simulink model "fullcar_7dof"  (R2026a)
settings: Solver=ode4  StopTime=t_end  FixedStep=dt
values from neighbouring files (symbols this model uses):
  Kfb = lqr(Aa, Ba, Q, R, N)    [controller_lqr.m]    (also in controller_skyhook.m = diag(c_sky) * [zeros(4, 7), veh.T, zeros(4, 4), zeros(4, 8)]; test_controllers.m = {zeros(4,22), K}; test_fullcar_model.m = K{1})
  x0 = -(A - Bu * Kfb(:, 1:14)) \ ((B(:, 5:12) - Bu * Kfb(:, 15:22)) * w(1, 2:9)')    [run_fullcar.m]    (also in test_fullcar_model.m = zeros(14,1))
undefined symbols (not defined in the file or in its folder): veh
settings Model: Creator=markn  LastModifiedBy=markn
settings DataIOCC: ExternalInput=w_in  LoadExternalInput=on
settings DebuggingCC: AlgebraicLoopMsg=error

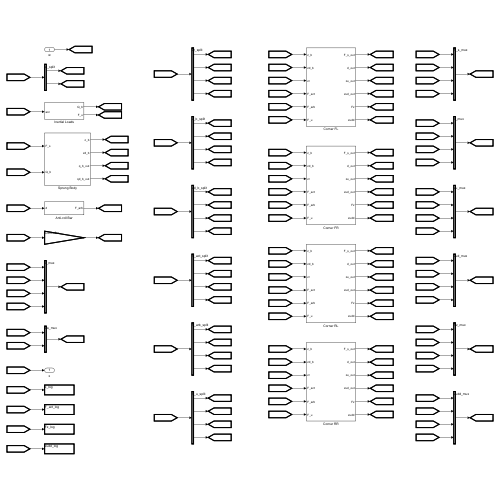
[thumbnail: Simulink's stored preview of the top-level diagram]
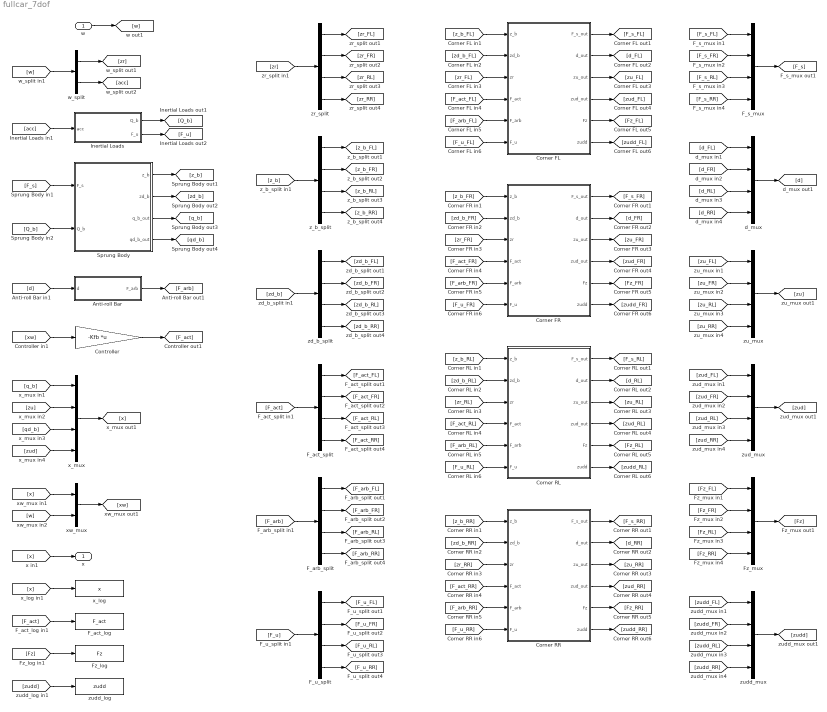
== system fullcar_7dof ==
  w : Inport  PortDimensions=8
  Anti-roll Bar : Subsystem
  Controller : Gain  Gain=-Kfb  Multiplication=Matrix(K*u)
  Corner FL : Subsystem
  Corner FR : Subsystem
  Corner RL : Subsystem
  Corner RR : Subsystem
  F_act_log : ToWorkspace  VariableName=F_act  SampleTime=-1
  F_act_split : Demux
  F_arb_split : Demux
  F_s_mux : Mux
  F_u_split : Demux
  Fz_log : ToWorkspace  VariableName=Fz  SampleTime=-1
  Fz_mux : Mux
  Inertial Loads : Subsystem
  Sprung Body : Subsystem
  d_mux : Mux
  w_split : Demux  Outputs=[4 4]
  x_log : ToWorkspace  VariableName=x  SampleTime=-1
  x_mux : Mux  Inputs=[3 4 3 4]
  xw_mux : Mux  Inputs=[14 8]
  z_b_split : Demux
  zd_b_split : Demux
  zr_split : Demux
  zu_mux : Mux
  zud_mux : Mux
  zudd_log : ToWorkspace  VariableName=zudd  SampleTime=-1
  zudd_mux : Mux
  x : Outport
  wires:
  w/1 -> [w]
  [w] -> w_split/1
  w_split/1 -> [zr]
  w_split/2 -> [acc]
  [acc] -> Inertial Loads/1(acc)
  Inertial Loads/1(Q_b) -> [Q_b]
  Inertial Loads/2(F_u) -> [F_u]
  [F_s] -> Sprung Body/1(F_s)
  [Q_b] -> Sprung Body/2(Q_b)
  Sprung Body/1(z_b) -> [z_b]
  Sprung Body/2(zd_b) -> [zd_b]
  Sprung Body/3(q_b_out) -> [q_b]
  Sprung Body/4(qd_b_out) -> [qd_b]
  [d] -> Anti-roll Bar/1(d)
  Anti-roll Bar/1(F_arb) -> [F_arb]
  [xw] -> Controller/1
  Controller/1 -> [F_act]
  [q_b] -> x_mux/1
  [zu] -> x_mux/2
  [qd_b] -> x_mux/3
  [zud] -> x_mux/4
  x_mux/1 -> [x]
  [x] -> xw_mux/1
  [w] -> xw_mux/2
  xw_mux/1 -> [xw]
  [x] -> x/1
  [x] -> x_log/1
  [F_act] -> F_act_log/1
  [Fz] -> Fz_log/1
  [zudd] -> zudd_log/1
  [zr] -> zr_split/1
  zr_split/1 -> [zr_FL]
  zr_split/2 -> [zr_FR]
  zr_split/3 -> [zr_RL]
  zr_split/4 -> [zr_RR]
  [z_b] -> z_b_split/1
  z_b_split/1 -> [z_b_FL]
  z_b_split/2 -> [z_b_FR]
  z_b_split/3 -> [z_b_RL]
  z_b_split/4 -> [z_b_RR]
  [zd_b] -> zd_b_split/1
  zd_b_split/1 -> [zd_b_FL]
  zd_b_split/2 -> [zd_b_FR]
  zd_b_split/3 -> [zd_b_RL]
  zd_b_split/4 -> [zd_b_RR]
  [F_act] -> F_act_split/1
  F_act_split/1 -> [F_act_FL]
  F_act_split/2 -> [F_act_FR]
  F_act_split/3 -> [F_act_RL]
  F_act_split/4 -> [F_act_RR]
  [F_arb] -> F_arb_split/1
  F_arb_split/1 -> [F_arb_FL]
  F_arb_split/2 -> [F_arb_FR]
  F_arb_split/3 -> [F_arb_RL]
  F_arb_split/4 -> [F_arb_RR]
  [F_u] -> F_u_split/1
  F_u_split/1 -> [F_u_FL]
  F_u_split/2 -> [F_u_FR]
  F_u_split/3 -> [F_u_RL]
  F_u_split/4 -> [F_u_RR]
  [z_b_FL] -> Corner FL/1(z_b)
  [zd_b_FL] -> Corner FL/2(zd_b)
  [zr_FL] -> Corner FL/3(zr)
  [F_act_FL] -> Corner FL/4(F_act)
  [F_arb_FL] -> Corner FL/5(F_arb)
  [F_u_FL] -> Corner FL/6(F_u)
  Corner FL/1(F_s_out) -> [F_s_FL]
  Corner FL/2(d_out) -> [d_FL]
  Corner FL/3(zu_out) -> [zu_FL]
  Corner FL/4(zud_out) -> [zud_FL]
  Corner FL/5(Fz) -> [Fz_FL]
  Corner FL/6(zudd) -> [zudd_FL]
  [z_b_FR] -> Corner FR/1(z_b)
  [zd_b_FR] -> Corner FR/2(zd_b)
  [zr_FR] -> Corner FR/3(zr)
  [F_act_FR] -> Corner FR/4(F_act)
  [F_arb_FR] -> Corner FR/5(F_arb)
  [F_u_FR] -> Corner FR/6(F_u)
  Corner FR/1(F_s_out) -> [F_s_FR]
  Corner FR/2(d_out) -> [d_FR]
  Corner FR/3(zu_out) -> [zu_FR]
  Corner FR/4(zud_out) -> [zud_FR]
  Corner FR/5(Fz) -> [Fz_FR]
  Corner FR/6(zudd) -> [zudd_FR]
  [z_b_RL] -> Corner RL/1(z_b)
  [zd_b_RL] -> Corner RL/2(zd_b)
  [zr_RL] -> Corner RL/3(zr)
  [F_act_RL] -> Corner RL/4(F_act)
  [F_arb_RL] -> Corner RL/5(F_arb)
  [F_u_RL] -> Corner RL/6(F_u)
  Corner RL/1(F_s_out) -> [F_s_RL]
  Corner RL/2(d_out) -> [d_RL]
  Corner RL/3(zu_out) -> [zu_RL]
  Corner RL/4(zud_out) -> [zud_RL]
  Corner RL/5(Fz) -> [Fz_RL]
  Corner RL/6(zudd) -> [zudd_RL]
  [z_b_RR] -> Corner RR/1(z_b)
  [zd_b_RR] -> Corner RR/2(zd_b)
  [zr_RR] -> Corner RR/3(zr)
  [F_act_RR] -> Corner RR/4(F_act)
  [F_arb_RR] -> Corner RR/5(F_arb)
  [F_u_RR] -> Corner RR/6(F_u)
  Corner RR/1(F_s_out) -> [F_s_RR]
  Corner RR/2(d_out) -> [d_RR]
  Corner RR/3(zu_out) -> [zu_RR]
  Corner RR/4(zud_out) -> [zud_RR]
  Corner RR/5(Fz) -> [Fz_RR]
  Corner RR/6(zudd) -> [zudd_RR]
  [F_s_FL] -> F_s_mux/1
  [F_s_FR] -> F_s_mux/2
  [F_s_RL] -> F_s_mux/3
  [F_s_RR] -> F_s_mux/4
  F_s_mux/1 -> [F_s]
  [d_FL] -> d_mux/1
  [d_FR] -> d_mux/2
  [d_RL] -> d_mux/3
  [d_RR] -> d_mux/4
  d_mux/1 -> [d]
  [zu_FL] -> zu_mux/1
  [zu_FR] -> zu_mux/2
  [zu_RL] -> zu_mux/3
  [zu_RR] -> zu_mux/4
  zu_mux/1 -> [zu]
  [zud_FL] -> zud_mux/1
  [zud_FR] -> zud_mux/2
  [zud_RL] -> zud_mux/3
  [zud_RR] -> zud_mux/4
  zud_mux/1 -> [zud]
  [Fz_FL] -> Fz_mux/1
  [Fz_FR] -> Fz_mux/2
  [Fz_RL] -> Fz_mux/3
  [Fz_RR] -> Fz_mux/4
  Fz_mux/1 -> [Fz]
  [zudd_FL] -> zudd_mux/1
  [zudd_FR] -> zudd_mux/2
  [zudd_RL] -> zudd_mux/3
  [zudd_RR] -> zudd_mux/4
  zudd_mux/1 -> [zudd]

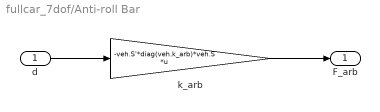
== system fullcar_7dof/Anti-roll Bar ==
  d : Inport
  k_arb : Gain  Gain=-veh.S'*diag(veh.k_arb)*veh.S  Multiplication=Matrix(K*u)
  F_arb : Outport
  wires:
  d/1 -> k_arb/1
  k_arb/1 -> F_arb/1

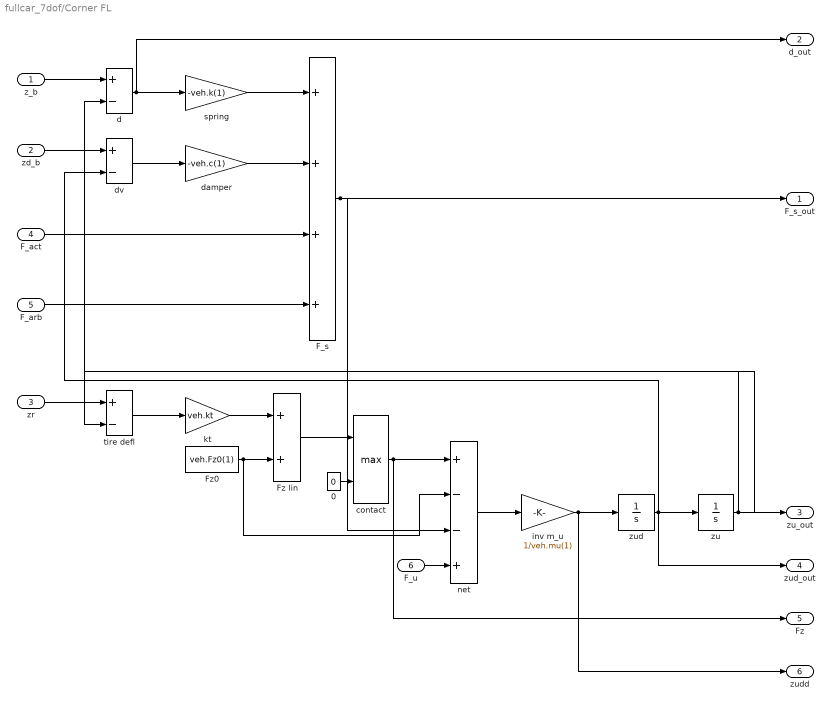
== system fullcar_7dof/Corner FL ==
  z_b : Inport
  zd_b : Inport  Port=2
  zr : Inport  Port=3
  F_act : Inport  Port=4
  F_arb : Inport  Port=5
  F_u : Inport  Port=6
  0 : Constant  Value=0
  F_s : Sum  Inputs=++++
  Fz lin : Sum
  Fz0 : Constant  Value=veh.Fz0(1)
  contact : MinMax  Function=max  Inputs=2
  d : Sum  Inputs=+-
  damper : Gain  Gain=-veh.c(1)
  dv : Sum  Inputs=+-
  inv m_u : Gain  Gain=1/veh.mu(1)
  kt : Gain  Gain=veh.kt
  net : Sum  Inputs=+--+
  spring : Gain  Gain=-veh.k(1)
  tire defl : Sum  Inputs=+-
  zu : Integrator  InitialCondition=x0(4)
  zud : Integrator  InitialCondition=x0(11)
  F_s_out : Outport
  d_out : Outport  Port=2
  zu_out : Outport  Port=3
  zud_out : Outport  Port=4
  Fz : Outport  Port=5
  zudd : Outport  Port=6
  wires:
  z_b/1 -> d/1
  zd_b/1 -> dv/1
  d/1 -> spring/1, d_out/1
  dv/1 -> damper/1
  spring/1 -> F_s/1
  damper/1 -> F_s/2
  F_act/1 -> F_s/3
  F_arb/1 -> F_s/4
  F_s/1 -> F_s_out/1, net/3
  zr/1 -> tire defl/1
  tire defl/1 -> kt/1
  kt/1 -> Fz lin/1
  Fz lin/1 -> contact/1
  contact/1 -> net/1, Fz/1
  net/1 -> inv m_u/1
  inv m_u/1 -> zud/1, zudd/1
  zud/1 -> zu/1, dv/2, zud_out/1
  Fz0/1 -> Fz lin/2, net/2
  0/1 -> contact/2
  F_u/1 -> net/4
  zu/1 -> d/2, tire defl/2, zu_out/1

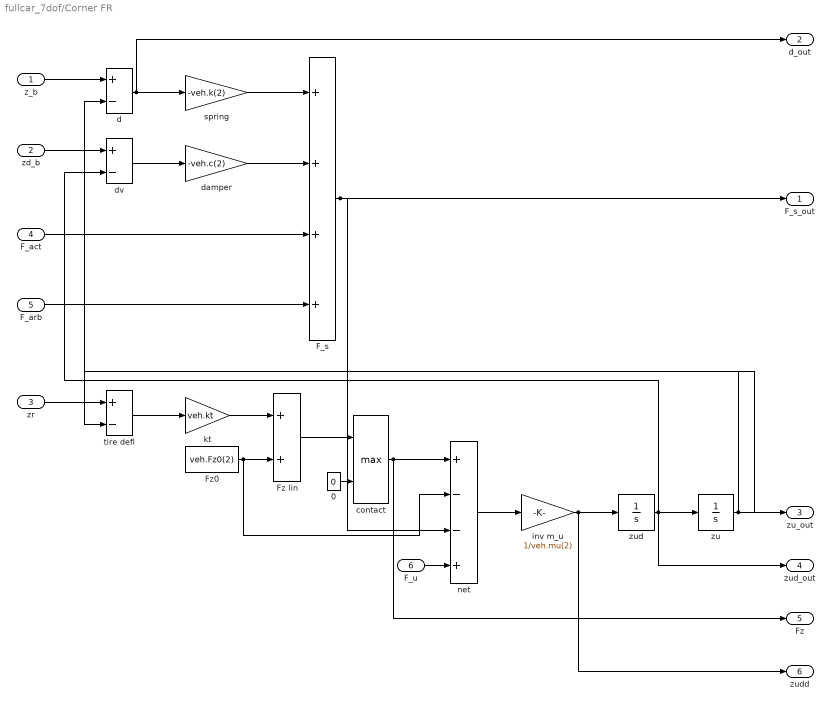
== system fullcar_7dof/Corner FR ==
  z_b : Inport
  zd_b : Inport  Port=2
  zr : Inport  Port=3
  F_act : Inport  Port=4
  F_arb : Inport  Port=5
  F_u : Inport  Port=6
  0 : Constant  Value=0
  F_s : Sum  Inputs=++++
  Fz lin : Sum
  Fz0 : Constant  Value=veh.Fz0(2)
  contact : MinMax  Function=max  Inputs=2
  d : Sum  Inputs=+-
  damper : Gain  Gain=-veh.c(2)
  dv : Sum  Inputs=+-
  inv m_u : Gain  Gain=1/veh.mu(2)
  kt : Gain  Gain=veh.kt
  net : Sum  Inputs=+--+
  spring : Gain  Gain=-veh.k(2)
  tire defl : Sum  Inputs=+-
  zu : Integrator  InitialCondition=x0(5)
  zud : Integrator  InitialCondition=x0(12)
  F_s_out : Outport
  d_out : Outport  Port=2
  zu_out : Outport  Port=3
  zud_out : Outport  Port=4
  Fz : Outport  Port=5
  zudd : Outport  Port=6
  wires:
  z_b/1 -> d/1
  zd_b/1 -> dv/1
  d/1 -> spring/1, d_out/1
  dv/1 -> damper/1
  spring/1 -> F_s/1
  damper/1 -> F_s/2
  F_act/1 -> F_s/3
  F_arb/1 -> F_s/4
  F_s/1 -> F_s_out/1, net/3
  zr/1 -> tire defl/1
  tire defl/1 -> kt/1
  kt/1 -> Fz lin/1
  Fz lin/1 -> contact/1
  contact/1 -> net/1, Fz/1
  net/1 -> inv m_u/1
  inv m_u/1 -> zud/1, zudd/1
  zud/1 -> zu/1, dv/2, zud_out/1
  Fz0/1 -> Fz lin/2, net/2
  0/1 -> contact/2
  F_u/1 -> net/4
  zu/1 -> d/2, tire defl/2, zu_out/1

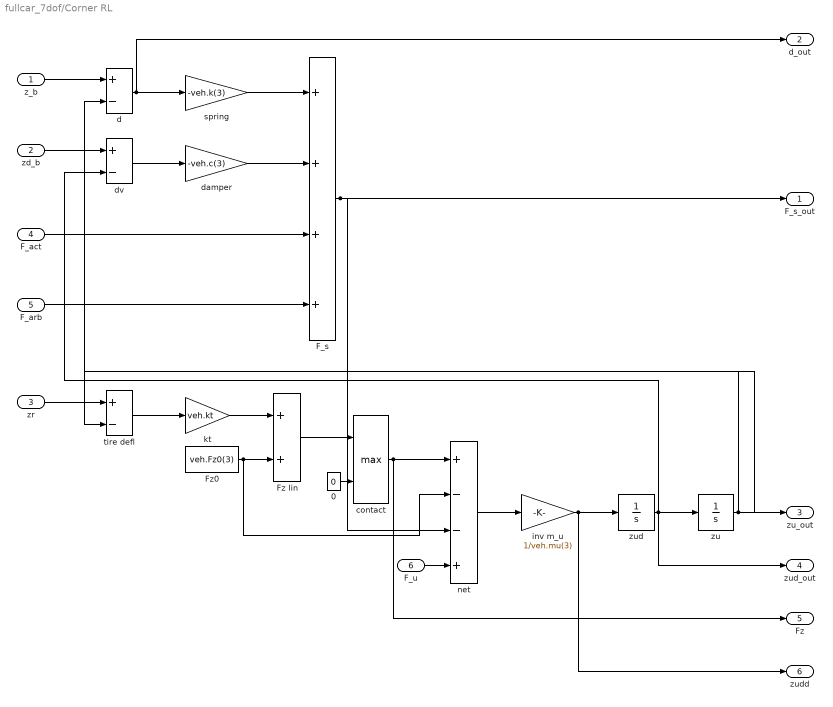
== system fullcar_7dof/Corner RL ==
  z_b : Inport
  zd_b : Inport  Port=2
  zr : Inport  Port=3
  F_act : Inport  Port=4
  F_arb : Inport  Port=5
  F_u : Inport  Port=6
  0 : Constant  Value=0
  F_s : Sum  Inputs=++++
  Fz lin : Sum
  Fz0 : Constant  Value=veh.Fz0(3)
  contact : MinMax  Function=max  Inputs=2
  d : Sum  Inputs=+-
  damper : Gain  Gain=-veh.c(3)
  dv : Sum  Inputs=+-
  inv m_u : Gain  Gain=1/veh.mu(3)
  kt : Gain  Gain=veh.kt
  net : Sum  Inputs=+--+
  spring : Gain  Gain=-veh.k(3)
  tire defl : Sum  Inputs=+-
  zu : Integrator  InitialCondition=x0(6)
  zud : Integrator  InitialCondition=x0(13)
  F_s_out : Outport
  d_out : Outport  Port=2
  zu_out : Outport  Port=3
  zud_out : Outport  Port=4
  Fz : Outport  Port=5
  zudd : Outport  Port=6
  wires:
  z_b/1 -> d/1
  zd_b/1 -> dv/1
  d/1 -> spring/1, d_out/1
  dv/1 -> damper/1
  spring/1 -> F_s/1
  damper/1 -> F_s/2
  F_act/1 -> F_s/3
  F_arb/1 -> F_s/4
  F_s/1 -> F_s_out/1, net/3
  zr/1 -> tire defl/1
  tire defl/1 -> kt/1
  kt/1 -> Fz lin/1
  Fz lin/1 -> contact/1
  contact/1 -> net/1, Fz/1
  net/1 -> inv m_u/1
  inv m_u/1 -> zud/1, zudd/1
  zud/1 -> zu/1, dv/2, zud_out/1
  Fz0/1 -> Fz lin/2, net/2
  0/1 -> contact/2
  F_u/1 -> net/4
  zu/1 -> d/2, tire defl/2, zu_out/1

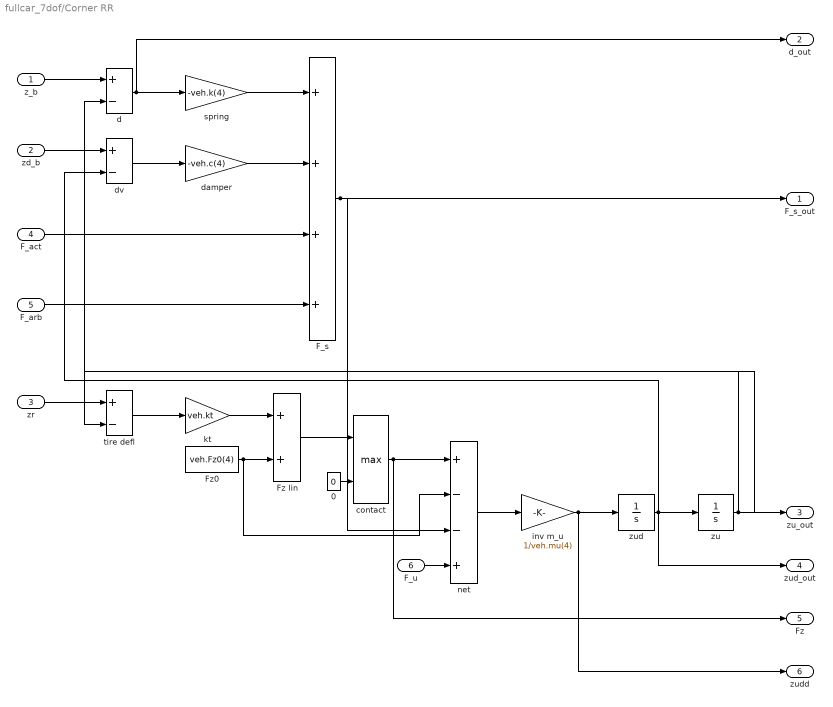
== system fullcar_7dof/Corner RR ==
  z_b : Inport
  zd_b : Inport  Port=2
  zr : Inport  Port=3
  F_act : Inport  Port=4
  F_arb : Inport  Port=5
  F_u : Inport  Port=6
  0 : Constant  Value=0
  F_s : Sum  Inputs=++++
  Fz lin : Sum
  Fz0 : Constant  Value=veh.Fz0(4)
  contact : MinMax  Function=max  Inputs=2
  d : Sum  Inputs=+-
  damper : Gain  Gain=-veh.c(4)
  dv : Sum  Inputs=+-
  inv m_u : Gain  Gain=1/veh.mu(4)
  kt : Gain  Gain=veh.kt
  net : Sum  Inputs=+--+
  spring : Gain  Gain=-veh.k(4)
  tire defl : Sum  Inputs=+-
  zu : Integrator  InitialCondition=x0(7)
  zud : Integrator  InitialCondition=x0(14)
  F_s_out : Outport
  d_out : Outport  Port=2
  zu_out : Outport  Port=3
  zud_out : Outport  Port=4
  Fz : Outport  Port=5
  zudd : Outport  Port=6
  wires:
  z_b/1 -> d/1
  zd_b/1 -> dv/1
  d/1 -> spring/1, d_out/1
  dv/1 -> damper/1
  spring/1 -> F_s/1
  damper/1 -> F_s/2
  F_act/1 -> F_s/3
  F_arb/1 -> F_s/4
  F_s/1 -> F_s_out/1, net/3
  zr/1 -> tire defl/1
  tire defl/1 -> kt/1
  kt/1 -> Fz lin/1
  Fz lin/1 -> contact/1
  contact/1 -> net/1, Fz/1
  net/1 -> inv m_u/1
  inv m_u/1 -> zud/1, zudd/1
  zud/1 -> zu/1, dv/2, zud_out/1
  Fz0/1 -> Fz lin/2, net/2
  0/1 -> contact/2
  F_u/1 -> net/4
  zu/1 -> d/2, tire defl/2, zu_out/1

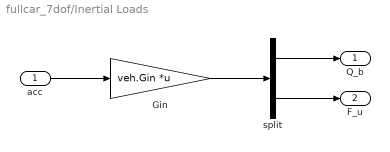
== system fullcar_7dof/Inertial Loads ==
  acc : Inport
  Gin : Gain  Gain=veh.Gin  Multiplication=Matrix(K*u)
  split : Demux  Outputs=[3 4]
  Q_b : Outport
  F_u : Outport  Port=2
  wires:
  acc/1 -> Gin/1
  Gin/1 -> split/1
  split/1 -> Q_b/1
  split/2 -> F_u/1

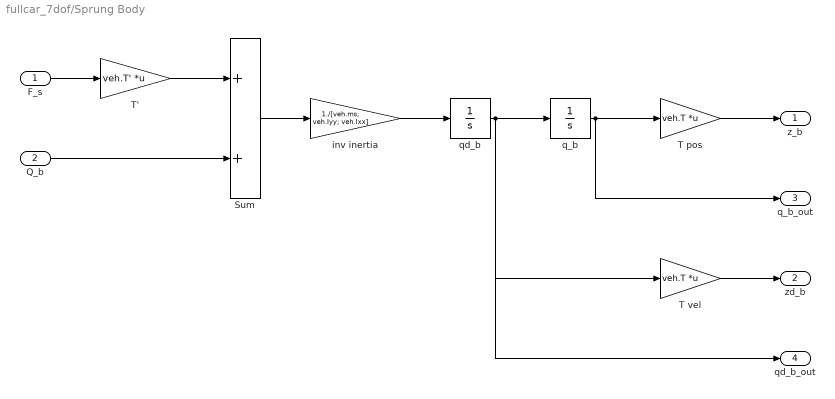
== system fullcar_7dof/Sprung Body ==
  F_s : Inport
  Q_b : Inport  Port=2
  Sum : Sum
  T pos : Gain  Gain=veh.T  Multiplication=Matrix(K*u)
  T vel : Gain  Gain=veh.T  Multiplication=Matrix(K*u)
  T' : Gain  Gain=veh.T'  Multiplication=Matrix(K*u)
  inv inertia : Gain  Gain=1./[veh.ms; veh.Iyy; veh.Ixx]
  q_b : Integrator  InitialCondition=x0(1:3)
  qd_b : Integrator  InitialCondition=x0(8:10)
  z_b : Outport
  zd_b : Outport  Port=2
  q_b_out : Outport  Port=3
  qd_b_out : Outport  Port=4
  wires:
  F_s/1 -> T'/1
  T'/1 -> Sum/1
  Q_b/1 -> Sum/2
  Sum/1 -> inv inertia/1
  inv inertia/1 -> qd_b/1
  qd_b/1 -> q_b/1, T vel/1, qd_b_out/1
  q_b/1 -> T pos/1, q_b_out/1
  T pos/1 -> z_b/1
  T vel/1 -> zd_b/1
